simulink model "StampFly_IMU400"  (R2026b)
settings: Solver=FixedStepDiscrete  StopTime=inf  FixedStep=Official.Step
PostLoadFcn:
  | run(fullfile(fileparts(get_param('StampFly_IMU400','FileName')),'config','startup.m'));
InitFcn:
  | init_imu_flight;
undefined symbols (not defined in the file): Bottom, Official
libraries: slpidlib x7, simulink x4, mspfiltlib x1
(part 4 of 4)

== matlab function StampFly_IMU400/AttitudeAltitudeEstimation400/IMUAttitude400/FilterInputs ==
  data: rates input; accelMps2 output; accelG input; mode input; reset input; gyroRps output; run output; filterReset output
function [accelMps2,gyroRps,run,filterReset]=IMUFilterInputs(rates,accelG,mode,reset)
%IMUFILTERINPUTS Match the previous estimator axes and use gravity-positive NED.
%#codegen
% The previous Madgwick frame is [bodyY bodyX -bodyZ]. Its accelerometer
% vector has +g on Z at rest. NED IMU Filter uses the same gravity sign.
accelMps2=single([accelG(2),accelG(1),-accelG(3)])*single(9.80665);
gyroRps=single([rates(2),rates(1),-rates(3)]);
run=mode>uint8(1);
% A disabled subsystem does not execute its Reset port. Retain reset requests
% during calibration/hold and apply them before the next fusion update.
persistent pendingReset
if isempty(pendingReset),pendingReset=false;end
if reset,pendingReset=true;end
filterReset=pendingReset;
if run,pendingReset=false;end
end

== matlab function StampFly_IMU400/AttitudeAltitudeEstimation400/IMUAttitude400/FlightOutputs ==
  data: orientation input; angles output; angularVelocity input; run input; reset input; rawRates input; q output; rates output
function [angles,q,rates]=IMUFlightOutputs(orientation,angularVelocity,run,reset,rawRates)
%IMUFLIGHTOUTPUTS Preserve the previous estimator's flight-facing conventions.
%#codegen
% Match the previous angle/quaternion hold behavior before estimation starts.
% A reset clears orientation but retains the last angles until the next update.
persistent heldAngles heldQuaternion heldBias
if isempty(heldAngles)
    heldAngles=zeros(3,1,'single');
    heldQuaternion=single([1;0;0;0]);
    heldBias=zeros(3,1,'single');
end
if reset
    heldQuaternion=single([1;0;0;0]);
    heldBias=zeros(3,1,'single');
end
correctedRates=single([angularVelocity(2);angularVelocity(1);-angularVelocity(3)]);
if run
    heldQuaternion=single(orientation(:));
    w=heldQuaternion(1);x=heldQuaternion(2);y=heldQuaternion(3);z=heldQuaternion(4);
    roll=atan2(single(2)*(w*x+y*z),single(1)-single(2)*(x*x+y*y));
    pitch=asin(min(single(1),max(single(-1),single(2)*(w*y-z*x))));
    yaw=atan2(single(2)*(x*y+w*z),single(1)-single(2)*(y*y+z*z));
    % Retain the original rounded radians/degrees factors and yaw offset.
    heldAngles=[pitch*single(57.29578);roll*single(57.29578); ...
        -(yaw*single(57.29578)+single(180))]*single(pi/180);
    heldBias=single(rawRates(:))-correctedRates;
end
angles=heldAngles;q=heldQuaternion;
% Keep the live gyro path when fusion is disabled; the retained residual bias
% is zero during startup and after reset. No extra sample delay is introduced.
rates=single(rawRates(:))-heldBias;
if run,rates=correctedRates;end
end

== stateflow chart StampFly_IMU400/FlightControl400/TakeoffHoverControl400/FlightCommand400/TakeoffLandingCommand ==
  settings: description=|
      | 離陸・ホバリング・着陸の指令生成（400 Hz）
      | Parking: 高度0.5 m/推力0へ初期化。自動離陸: 0〜499周期は3.8 V基準、500〜999周期は実電圧トリム。
      | AutoHover: 1000周期後の基準推力。目標高度0.05〜1.8 m、スティックで更新。
      | ManualAltitude/AutoHover/Landingの遷移条件は図に表示。演算順・状態保持・AltFlag保持は公式互換。
      | Chart内にMATLAB関数は置かない。
  state CommandPhases [parallel]
    settings: executionOrder=1
    state Parking
      en: Base=single(0);Alt=single(.5);Counter=uint16(0);landingActive=false;AltFlag=false;
    state TakeoffReference
      en: ControlMode=uint8(stick(5));AltFlag=true;
      Base=min(single(Counter)/single(1000),(-single(.2448)*single(3.8)+single(1.5892)));Counter=Counter+uint16(1);
      th=stick(4);if th>-.2 && th<.2,th=single(0);end
      Alt=min(max(single(double(Alt)+double(th)*.001),single(.05)),single(1.8));
      if rangeFlag>RangeOld || rangeFlag==20,Base=Base-single(.02);RangeOld=rangeFlag;end
      raw=single(double(Base)*3.7);
    state ManualAltitude
      en: ControlMode=uint8(stick(5));manual=true;th=min(max(stick(4),single(0)),single(1));
      if th>-.2 && th<.2,th=single(0);end
      raw=single((.00413+double(single(3.3)*th-single(5.44)*th*th+single(3.13)*th*th*th))*3.7);
    state TakeoffBattery
      en: ControlMode=uint8(stick(5));AltFlag=true;
      Base=min(single(Counter)/single(1000),(-single(.2448)*voltage+single(1.5892)));Counter=Counter+uint16(1);
      th=stick(4);if th>-.2 && th<.2,th=single(0);end
      Alt=min(max(single(double(Alt)+double(th)*.001),single(.05)),single(1.8));
      if rangeFlag>RangeOld || rangeFlag==20,Base=Base-single(.02);RangeOld=rangeFlag;end
      raw=single(double(Base)*3.7);
    state AutoHover
      en: ControlMode=uint8(stick(5));AltFlag=true;
      Base=(-single(.2448)*voltage+single(1.5892));
      th=stick(4);if th>-.2 && th<.2,th=single(0);end
      Alt=min(max(single(double(Alt)+double(th)*.001),single(.05)),single(1.8));
      if rangeFlag>RangeOld || rangeFlag==20,Base=Base-single(.02);RangeOld=rangeFlag;end
      raw=single(double(Base)*3.7);
    state Landing
      en: AltFlag=false;
      if ~landingActive,landingActive=true;History(:)=height;Base=(-single(.2448)*voltage+single(1.5892));end
      if History(10)>=height,Base=single(double(Base)*.9999);end
      if height<.15,Base=single(double(Base)*.999);end
      if height<.1,landingActive=false;end
      for j=2:10,History(j)=History(j-1);end
      History(1)=height;
    state Hold
    CommandPhases -> (junction 50) : step
    (junction 50) -> AutoHover [order 6] : [mode==2 && uint8(stick(6))==4]
    (junction 50) -> Hold [order 7]
    (junction 50) -> Parking [order 1] : [mode==3]
    (junction 50) -> Landing [order 2] : [mode==5]
    (junction 50) -> TakeoffBattery [order 5] : [mode==2 && uint8(stick(6))==4 && Counter<1000]
    (junction 50) -> TakeoffReference [order 4] : [mode==2 && uint8(stick(6))==4 && Counter<500]
    (default) -> Hold : /{Alt=single(.5);Base=single(0);Counter=uint16(0);RangeOld=uint8(0);landingActive=false;History=zeros(10,1,'single');AltFlag=false;ControlMode=uint8(0);th=single(0);j=double(0);}
    (junction 50) -> ManualAltitude [order 3] : [mode==2 && uint8(stick(6))~=4]
  state CycleOutputs [parallel]
    en: raw=single(0);manual=false;
    send(step,CommandPhases);
    alt=Alt;base=Base;counter=Counter;auto=AltFlag;controlMode=single(ControlMode);
    du: raw=single(0);manual=false;
    send(step,CommandPhases);
    alt=Alt;base=Base;counter=Counter;auto=AltFlag;controlMode=single(ControlMode);
    settings: executionOrder=2
  note: 離陸・ホバリング・着陸の指令生成（400 Hz）
      | Parking: 高度0.5 m/推力0へ初期化。自動離陸: 0〜499周期は3.8 V基準、500〜999周期は実電圧トリム。
      | AutoHover: 1000周期後の基準推力。目標高度0.05〜1.8 m、スティックで更新。
      | ManualAltitude/AutoHover/Landingの遷移条件は図に表示。演算順・状態保持・AltFlag保持は公式互換。
      | Chart内にMATLAB関数は置かない。
  data: stick input single; height input single; voltage input single; rangeFlag input uint8; mode input uint8; alt output single; base output single; counter output uint16; raw output single; auto output boolean; manual output boolean; controlMode output single; Alt local single; Base local single; Counter local uint16; RangeOld local uint8; landingActive local boolean; History local single; AltFlag local boolean; ControlMode local uint8; th local single; j local double
  events: step local FUNCTION_CALL_EVENT

== matlab function StampFly_IMU400/LEDAndBuzzer400/StatusOutputs400/StatusIndicators400 ==
  data: arg_mode input uint8; arg_color1 output uint32; arg_controlMode input single; arg_altFlag input uint8; arg_lowVoltage input uint8; arg_rcError input uint8; arg_ahrsFlag input uint8; arg_button input uint8; arg_color2 output uint32; arg_tone output uint32; arg_restart output boolean
function [arg_color1,arg_color2,arg_tone,arg_restart]=stepFn(arg_mode,arg_controlMode,arg_altFlag,arg_lowVoltage,arg_rcError,arg_ahrsFlag,arg_button)
% 公式led_driveの状態色。ブザーの200ms待機は400Hzカウンターへ置換。
%#codegen
persistent Blink Rainbow C1 C2 Tick AHRSPrev ToneTicks ButtonCount WasPressed;
if isempty(Blink)
 Blink=uint16(0);Rainbow=uint32(255);C1=uint32(0);C2=uint32(0);Tick=uint16(0);AHRSPrev=uint8(0);ToneTicks=uint16(0);ButtonCount=uint8(0);WasPressed=false;
end
if arg_mode==1,C1=uint32(hex2dec('FF00FF'));C2=C1;
elseif arg_mode==5,C1=uint32(hex2dec('00FF00'));C2=C1;
elseif arg_mode==2
 c=uint32(hex2dec('FFFF00'));
 if arg_controlMode~=0,c=uint32(hex2dec('DC669B'));end
 if arg_altFlag>=1,c=uint32(hex2dec('331155'));end
 if arg_rcError==1,c=uint32(hex2dec('FF0000'));end
 C1=c;C2=c;if arg_lowVoltage>=100,C1=uint32(hex2dec('18EBF9'));end
elseif arg_mode==3
 if arg_lowVoltage<100
  if Blink==0
   top=bitand(Rainbow,uint32(hex2dec('800000')))~=0;Rainbow=bitshift(Rainbow,1);if top,Rainbow=bitor(Rainbow,uint32(1));end
   C1=Rainbow;C2=Rainbow;Blink=Blink+uint16(1);
  end
  Blink=Blink+uint16(1);if Blink>20,Blink=uint16(0);end
 else
  if Blink<10,C1=uint32(hex2dec('18EBF9'));C2=C1;
  elseif Blink<200,C1=uint32(0);C2=uint32(0);else,Blink=uint16(0);end
  Blink=Blink+uint16(1);
 end
 if arg_ahrsFlag~=AHRSPrev && arg_ahrsFlag==1,ToneTicks=uint16(80);end
 AHRSPrev=arg_ahrsFlag;
end
arg_tone=uint32(0);
% Startup notes from official buzzer.h. Four 200ms notes, then silence.
if Tick<320
 notes=uint32([294 441 350 393]);idx=min(floor(double(Tick)/80)+1,4);arg_tone=notes(idx);Tick=Tick+uint16(1);
elseif ToneTicks>0,arg_tone=uint32(4000);ToneTicks=ToneTicks-uint16(1);end
arg_restart=false;
if arg_button==1,ButtonCount=min(ButtonCount+uint8(1),uint8(40));if ButtonCount>=4,WasPressed=true;end
elseif WasPressed,arg_restart=true;WasPressed=false;ButtonCount=uint8(0);else,ButtonCount=uint8(0);end
% FastLED brightness15, show32: cap displayed channels without changing logic.
arg_color1=scale(C1);arg_color2=scale(C2);
end
function c=scale(x)
r=bitand(bitshift(x,-16),uint32(255));g=bitand(bitshift(x,-8),uint32(255));b=bitand(x,uint32(255));
c=bitor(bitor(bitshift(uint32(double(r)*15/255),16),bitshift(uint32(double(g)*15/255),8)),uint32(double(b)*15/255));
end

== matlab function StampFly_IMU400/FlightControl400/TakeoffHoverControl400/AltitudeControl400/SelectVerticalReference ==
  data: arg_zRef input single; arg_vRef output single; arg_mode input uint8; arg_auto input boolean
function arg_vRef=stepFn(arg_zRef,arg_mode,arg_auto)
% Auto高度補正が優先。公式else-ifの順序を維持。
%#codegen
arg_vRef=arg_zRef;if ~arg_auto && arg_mode==5,arg_vRef=single(-.15);end
end

== matlab function StampFly_IMU400/JoystickFeedback40/JoyStickTelemetry40/OfficialTelemetryValues ==
  data: arg_t input single; arg_values output single; arg_dt input single; arg_a input single; arg_r input single; arg_cd input single; arg_accel input single; arg_voltage input single; arg_duty input single; arg_z input single; arg_sd input single; arg_v input single
function arg_values=stepFn(arg_t,arg_dt,arg_a,arg_r,arg_cd,arg_accel,arg_voltage,arg_duty,arg_z,arg_sd,arg_v)
% 公式120byteテレメトリの27個のfloat。バイト送信は専用IOブロック。
%#codegen
arg_values=zeros(27,1,'single');arg_values(1:2)=[arg_t;arg_dt];arg_values(3:8)=[arg_a;arg_r]*single(180/pi);
arg_values(9:13)=arg_cd(6:10)*single(180/pi);arg_values(14)=single(double(arg_cd(5))/3.7);
arg_values(15)=arg_voltage;arg_values(16:18)=arg_accel([2 1 3])/single(9.80665);arg_values(18)=-arg_values(18);
arg_values(19:20)=[arg_v;arg_cd(4)];arg_values(21:22)=arg_duty(2:3);
arg_values(23:27)=[arg_cd(1);arg_z;arg_sd(3);arg_sd(1:2)];
end

== matlab function StampFly_IMU400/FlightControl400/TakeoffHoverControl400/AltitudeControl400/ThrustCorrectionLimits ==
  data: arg_arg_command input single; arg_arg_thrust output single; arg_arg_correction input single; arg_arg_base input single; arg_arg_auto input boolean; arg_arg_manual input boolean; arg_arg_velEnable input boolean; arg_branch input uint8; arg_arg_dt input single; arg_arg_oldFilter input single; arg_arg_lastThrust input single; arg_arg_filter output single; arg_arg_last output single
function [arg_arg_thrust,arg_arg_filter,arg_arg_last]=stepFn(arg_arg_command,arg_arg_correction,arg_arg_base,arg_arg_auto,arg_arg_manual,arg_arg_velEnable,arg_branch,arg_arg_dt,arg_arg_oldFilter,arg_arg_lastThrust)
% Auto correction takes priority over landing correction.
%#codegen
arg_arg_thrust=arg_arg_command;arg_arg_filter=arg_arg_oldFilter;
if arg_branch==3,arg_arg_filter=single(0);elseif arg_arg_manual,arg_arg_filter=arg_arg_command;end
if arg_arg_velEnable
 arg_arg_filter=filterStep(single(double(arg_arg_base+arg_arg_correction)*3.7),arg_arg_dt,single(.01),arg_arg_filter);arg_arg_thrust=arg_arg_filter;
 if arg_arg_auto
  if double(arg_arg_thrust)/3.7>double(single(arg_arg_base*single(1.15))),arg_arg_thrust=single(3.7*double(arg_arg_base)*double(single(1.15)));end
  if double(arg_arg_thrust)/3.7<double(single(arg_arg_base*single(.85))),arg_arg_thrust=single(3.7*double(arg_arg_base)*double(single(.85)));end
 end
end
if arg_branch==3,arg_arg_thrust=arg_arg_lastThrust;arg_arg_last=arg_arg_lastThrust;else,arg_arg_last=arg_arg_thrust;end
end
function s=filterStep(u,h,T,s),s=s*T/(T+h)+u*h/(T+h);end

== matlab function StampFly_IMU400/FlightControl400/TakeoffHoverControl400/AttitudeControl400/StickToAngleRate ==
  data: arg_arg_stick input single; arg_arg_angle output single; arg_branch input uint8; arg_arg_run input boolean; arg_arg_reset input boolean; arg_arg_lastRate input single; arg_arg_controlMode input single; arg_arg_directRate output single; arg_arg_resetError output single
function [arg_arg_angle,arg_arg_directRate,arg_arg_resetError]=stepFn(arg_arg_stick,arg_branch,arg_arg_run,arg_arg_reset,arg_arg_lastRate,arg_arg_controlMode)
% command、角度目標、中立点を別々に保持。Sportは角度commandを更新しない。
%#codegen
persistent Angle Centers AngleCmd YawCmd;
if isempty(Angle),Angle=zeros(2,1,'single');Centers=zeros(3,1,'single');AngleCmd=zeros(2,1,'single');YawCmd=single(0);end
arg_arg_directRate=arg_arg_lastRate;arg_arg_resetError=Angle;
commandCalled=arg_branch==2 || arg_branch==5;
if commandCalled
 if uint8(arg_arg_controlMode)==0 || arg_branch==5,AngleCmd=min(max(single(.4*double(arg_arg_stick(1:2))),single(-1)),single(1));end
 YawCmd=min(max(arg_arg_stick(3),single(-1)),single(1));
 arg_arg_directRate(3)=single(2*pi*double(YawCmd-Centers(3)));
 if uint8(arg_arg_controlMode)==1,arg_arg_directRate(1)=rateCommand(arg_arg_stick(1));arg_arg_directRate(2)=rateCommand(arg_arg_stick(2));end
end
if arg_arg_reset,Centers(1:2)=AngleCmd;end
if arg_arg_reset,Centers(3)=YawCmd;end
if arg_arg_run && uint8(arg_arg_controlMode)==0
 limit=single(30*pi/180);Angle=min(max(single(.5*pi*double(AngleCmd-Centers(1:2))),-limit),limit);
end
if arg_branch==3,arg_arg_directRate(1)=single(0);end
if arg_arg_reset,arg_arg_directRate(:)=single(0);end
arg_arg_angle=Angle;
end
function y=rateCommand(x)
x=min(max(x,single(-1)),single(1));a=abs(x);t=a*(a*a*a*a*a*single(.5)+a*single(.5));
y=single(pi/180)*((single(1600)-single(70))*t+single(70)*a);if x<0,y=-y;end
end

== matlab function StampFly_IMU400/FlightControl400/TakeoffHoverControl400/AttitudeControl400/SelectRateReference ==
  data: direct input single; rate output single; rollPID input single; pitchPID input single; angleEnable input boolean
function rate =stepFn(direct,rollPID,pitchPID,angleEnable)
% 日本語の説明はブロック注釈とDescriptionを参照。
%#codegen
            rate=direct;if angleEnable,rate(1)=rollPID;rate(2)=pitchPID;end
end

== matlab function StampFly_IMU400/FlightControl400/TakeoffHoverControl400/FlightDiagnostics400/ControlDiagnosticPack ==
  data: alt input single; diag output single; base input single; counter input uint16; zRef input single; thrust input single; angle input single; rate input single; rollTorque input single; pitchTorque input single; yawTorque input single; before input single
function diag =stepFn(alt,base,counter,zRef,thrust,angle,rate,rollTorque,pitchTorque,yawTorque,before)
% 日本語の説明はブロック注釈とDescriptionを参照。
%#codegen
            diag=[alt;base;single(counter);zRef;thrust;angle;rate;rollTorque;pitchTorque;yawTorque;before];
end

== stateflow chart StampFly_IMU400/FlightControl400/TakeoffHoverControl400/FlightCommand400/FinalizeFlightMode ==
  settings: description=Normal flight: finalize the mode; excessive acceleration and completed landing return to parking.
  state FinalModes [parallel]
    settings: executionOrder=1
    state OTHER
      en: mode=preMode;
    state INIT
      en: mode=uint8(0);
    state LANDING
      en: mode=uint8(5);
    state PARKING
      en: mode=uint8(3);
    state FLIGHT
      en: mode=uint8(2);
    state AVERAGE
      en: mode=uint8(1);
    (default) -> INIT
    (junction 27) -> OTHER [order 8]
    (junction 27) -> INIT [order 3] : [preMode==uint8(0)]
    FinalModes -> (junction 27) : decide
    (junction 27) -> AVERAGE [order 4] : [preMode==uint8(1)]
    (junction 27) -> LANDING [order 7] : [preMode==uint8(5)]
    (junction 27) -> FLIGHT [order 6] : [preMode==uint8(2)]
    (junction 27) -> PARKING [order 5] : [preMode==uint8(3)]
    (junction 27) -> PARKING [order 2] : [branch==5 && height<.1]
    (junction 27) -> PARKING [order 1] : [(branch==2 || branch==5) && overG==1]
  state CycleInput [parallel]
    en: mode=preMode;send(decide,FinalModes);
    du: mode=preMode;send(decide,FinalModes);
    settings: executionOrder=2
  note: Basic flight: takeoff, hover, landing and normal fault handling.
  data: branch input uint8; preMode input uint8; height input single; overG input uint8; mode output uint8
  events: decide local FUNCTION_CALL_EVENT

== matlab function StampFly_IMU400/FlightControl400/TakeoffHoverControl400/FlightCommand400/ControlGating400/ControlEnableReset ==
  data: arg_arg_raw input single; arg_arg_command output single; arg_arg_manual input boolean; arg_arg_auto input boolean; arg_branch input uint8; arg_arg_controlMode input single; arg_arg_dt input single; arg_arg_oldFilter input single; arg_arg_lastThrust input single; arg_arg_mode input uint8; arg_arg_run output boolean; arg_arg_reset output boolean; arg_arg_altEnable output boolean; arg_arg_angleEnable output boolean; arg_arg_velEnable output boolean
function [arg_arg_command,arg_arg_run,arg_arg_reset,arg_arg_altEnable,arg_arg_angleEnable,arg_arg_velEnable]=stepFn(arg_arg_raw,arg_arg_manual,arg_arg_auto,arg_branch,arg_arg_controlMode,arg_arg_dt,arg_arg_oldFilter,arg_arg_lastThrust,arg_arg_mode)
% Normal-flight enable/reset decisions and thrust filtering.
%#codegen
arg_arg_command=arg_arg_raw;
if arg_arg_manual,arg_arg_command=filterStep(arg_arg_raw,arg_arg_dt,single(.01),arg_arg_oldFilter);end
if arg_branch==5 || arg_branch==3,arg_arg_command=arg_arg_lastThrust;end
active=arg_branch==2 || arg_branch==5;
arg_arg_reset=active && double(arg_arg_command)/3.7<double(single(.1));
arg_arg_run=active && ~arg_arg_reset;
arg_arg_altEnable=arg_arg_run && arg_arg_auto;
arg_arg_angleEnable=arg_arg_run && uint8(arg_arg_controlMode)==0;
arg_arg_velEnable=arg_arg_run && (arg_arg_auto || arg_arg_mode==5);
end
function s=filterStep(u,h,T,s),s=s*T/(T+h)+u*h/(T+h);end

== matlab function StampFly_IMU400/SensorCorrection400/IMUBiasCalibration ==
  data: a input single; offset output single; g input single; mode input uint8; count output uint16
function [offset,count]=stepFn(a,g,mode)
% 日本語の説明はブロック注釈とDescriptionを参照。
%#codegen
persistent Offset Count;
if isempty(Offset)
Offset=zeros(4,1,'single');
Count=uint16(0);
end
            if mode==0,Offset(:)=single(0);Count=uint16(0);
            elseif mode==1 && Count<uint16(800)
                n=single(Count);
                Offset=(n*Offset+[g;a(3)])/(n+single(1));
                Count=Count+uint16(1);
            end
            offset=Offset;count=Count;
end

== matlab function StampFly_IMU400/SensorCorrection400/ToFHoldOutlierFilter ==
  data: mm input int16; alt output single; fresh input uint8; mode input uint8; dt input single; raw output int16
function [alt,raw]=stepFn(mm,fresh,mode,dt)
% 日本語の説明はブロック注釈とDescriptionを参照。
%#codegen
persistent History Range Raw Outlier Alt PreviousMode;
if isempty(History)
History=zeros(4,1,'int16');
Range=int16(0);
Raw=int16(0);
Outlier=uint8(0);
Alt=single(0);
PreviousMode=uint8(0);
end
            if mode==3 && mode~=PreviousMode,History(:)=int16(0);Alt=single(0);end
            if mode>1
                if fresh~=0
                    Raw=mm;if mm>int16(20),Range=mm;end
                    delta=int32(Range)-int32(History(2));
                    if abs(delta)>int32(500) && Outlier<uint8(2)
                        extrap=int32(History(2))+idivide(int32(History(2))-int32(History(4)),int32(2),'fix');
                        Range=int16(extrap);Outlier=Outlier+uint8(1);
                    else
                        Outlier=uint8(0);History(4)=History(3);History(3)=History(2);History(2)=Range;
                    end
                end
                Alt=filterStep(single(double(Range)/1000),dt,single(0.005),Alt);
            end
            alt=Alt;raw=Raw;PreviousMode=mode;
end

function s = filterStep(u,h,T,s)
%FILTERSTEP Exact Filter::update, including operation ordering.
%#codegen
s = s*T/(T+h) + u*h/(T+h);
end

== matlab function StampFly_IMU400/AttitudeAltitudeEstimation400/AltitudeKalman ==
  data: alt input single; height output single; az input single; mode input uint8; dt input single; parkingReset input boolean; velocity output single; bias output single
function [height,velocity,bias]=stepFn(alt,az,mode,dt,parkingReset)
% 日本語の説明はブロック注釈とDescriptionを参照。
%#codegen
persistent State First PreviousMode;
if isempty(State)
State=kalmanInitial();
First=false;
PreviousMode=uint8(0);
end
            if parkingReset,[~,State]=kalmanStep(single(0),single(0),dt,true,State);end
            if mode==3 && mode~=PreviousMode,First=false;end
            if mode>1
                if First,[~,State]=kalmanStep(alt,az,dt,false,State);else,First=true;end
            end
            velocity=State.output(1);height=State.output(2);bias=State.output(3);PreviousMode=mode;
end

function [y,s] = kalmanStep(z,acc,h,resetState,s)
%KALMANSTEP Direct translation of Alt_kalman::update, state [v;z;bias].
% Preserve reset(): covariance and public output reset, private x is retained.
%#codegen
if resetState
    s.P = single(100)*eye(3,'single'); s.output(:) = single(0);
else
    p=s.P; b=single(-0.01); f=single(1)+h*b;
    xp=[s.x(1)+(acc-s.x(3))*h;s.x(2)+s.x(1)*h;s.x(3)*f];
    pp=zeros(3,3,'single');
    pp(1,1)=p(1,1)-h*(p(3,1)+p(1,3))+h*h*p(3,3)+h*h*single(0.01);
    pp(1,2)=h*(p(1,1)-p(3,2))-h*h*p(3,1)+p(1,2);
    pp(1,3)=f*(p(1,3)-h*p(3,3));
    pp(2,1)=h*(p(1,1)-p(2,3))-h*h*p(1,3)+p(2,1);
    pp(2,2)=h*h*p(1,1)+h*(p(2,1)+p(1,2))+p(2,2);
    pp(2,3)=f*(p(2,3)+h*p(1,3));
    pp(3,1)=f*(p(3,1)-h*p(3,3));
    pp(3,2)=f*(p(3,2)+h*p(3,1));
    pp(3,3)=f*f*p(3,3)+h*h;
    k=[pp(1,2);pp(2,2);pp(3,2)]/(pp(2,2)+single(0.004*0.004));
    e=z-xp(2); s.x=xp+k*e; s.output=s.x;
    s.P(1,:)=pp(1,:)-k(1)*pp(2,:);
    s.P(2,:)=pp(2,:)*(single(1)-k(2));
    s.P(3,:)=-k(3)*pp(2,:)+pp(3,:);
end
y=s.output;
end

function s = kalmanInitial()
%#codegen
s = struct('x',zeros(3,1,'single'),'P',single(100)*eye(3,'single'), ...
    'output',zeros(3,1,'single'));
end

== matlab function StampFly_IMU400/AttitudeAltitudeEstimation400/SensorFlags ==
  data: arg_accel input single; arg_flags output uint8; arg_azd input single; arg_voltage input single; arg_mode input uint8; arg_altFlag input uint8; arg_height input single; arg_rawRange input int16; arg_dt input single; arg_parkingReset input boolean
function arg_flags =stepFn(arg_accel,arg_azd,arg_voltage,arg_mode,arg_altFlag,arg_height,arg_rawRange,arg_dt,arg_parkingReset)
% 日本語の説明はブロック注釈とDescriptionを参照。
%#codegen
persistent Norm Voltage OverG RangeFlag LowVoltage PreviousMode;
if isempty(Norm)
Norm=single(0);
Voltage=single(0);
OverG=uint8(0);
RangeFlag=uint8(0);
LowVoltage=uint8(0);
PreviousMode=uint8(0);
end
            if arg_parkingReset,OverG=uint8(0);RangeFlag=uint8(0);end
            if arg_mode==3 && arg_mode~=PreviousMode,Norm=single(0);end
            if arg_mode>1
                if (arg_height>single(2) && arg_altFlag~=0) || arg_rawRange==0,RangeFlag=min(RangeFlag+uint8(1),uint8(20));else,RangeFlag=uint8(0);end
            end
            normA=sqrt(arg_accel(1)*arg_accel(1)+arg_accel(2)*arg_accel(2)+arg_azd*arg_azd);
            Norm=filterStep(normA,arg_dt,single(.005),Norm);
            if Norm>single(2),OverG=uint8(1);end
            Voltage=filterStep(arg_voltage,arg_dt,single(.005),Voltage);
            if LowVoltage~=uint8(100)
                if Voltage<single(3.34),LowVoltage=LowVoltage+uint8(1);else,LowVoltage=uint8(0);end
                LowVoltage=min(LowVoltage,uint8(100));
            end
            arg_flags=[OverG;RangeFlag;LowVoltage];PreviousMode=arg_mode;
end

function s = filterStep(u,h,T,s)
%FILTERSTEP Exact Filter::update, including operation ordering.
%#codegen
s = s*T/(T+h) + u*h/(T+h);
end

== stateflow chart StampFly_IMU400/OfficialFlightSupervisor ==
  settings: description=|
      | 飛行モードの状態遷移図（400 Hz）
      | INIT→AVERAGE→PARKING→FLIGHT→LANDING。通信途絶・OverG・ボタンを遷移条件で判断。
      | CycleInputsが1周期分の入力を整理し、syncで前周期の確定状態に同期、decideで今回の遷移を実行。
      | branchは今回の分岐開始状態、modeは今回の判断後の状態。MATLAB関数はChart内に置かない。
  state FlightModes [parallel]
    settings: executionOrder=1
    state PARKING
      en: mode=uint8(3);
    state AVERAGE
      en: mode=uint8(1);
    state INIT
      en: mode=uint8(0);
    state FLIGHT
      en: mode=uint8(2);
    state LANDING
      en: mode=uint8(5);
    state OTHER
      en: mode=branch;
    (default) -> INIT : /{calibration=uint16(0); buttonCounter=int8(0); buttonState=uint8(0); chatter=uint8(0); lastAHRS=uint8(0); connectionCounter=uint16(0); buttonEvent=false; calibrationDone=false;}
    AVERAGE -> PARKING : decide[calibrationDone]
    INIT -> AVERAGE : decide
    (junction 43) -> AVERAGE [order 2] : [branch==uint8(1)]
    (junction 43) -> INIT [order 1] : [branch==uint8(0)]
    PARKING -> FLIGHT : decide[buttonEvent]/{ahrsReset=true;}
    FLIGHT -> PARKING [order 1] : decide[flags(1)==1]/{ahrsReset=true;}
    (junction 43) -> PARKING [order 3] : [branch==uint8(3)]
    LANDING -> PARKING : decide[buttonEvent]
    FLIGHT -> LANDING [order 2] : decide[buttonEvent || connected==0]/{ahrsReset=true;}
    (junction 43) -> LANDING [order 5] : [branch==uint8(5)]
    (junction 43) -> FLIGHT [order 4] : [branch==uint8(2)]
    FlightModes -> (junction 43) : sync
    (junction 43) -> OTHER [order 6]
  state CycleInputs [parallel]
    en: branch=previousMode; mode=branch; ahrsReset=false; parkingReset=branch==3;
    buttonEvent=false; calibrationDone=false;
    if newPacket~=0, connectionCounter=uint16(0); end
    connected=uint8(connectionCounter<uint16(40));
    if branch==1
    calibrationDone=calibration>=uint16(800);
    if ~calibrationDone, calibration=calibration+uint16(1); end
    elseif branch~=0
    if button==1
    buttonCounter=buttonCounter+int8(1);
    if buttonCounter>int8(10),buttonCounter=int8(10);buttonState=uint8(1);end
    else
    buttonCounter=buttonCounter-int8(1);
    if buttonCounter<int8(-10),buttonCounter=int8(-10);buttonState=uint8(0);end
    end
    if chatter==0
    if buttonState==1,chatter=uint8(1);end
    elseif buttonState==0
    chatter=chatter+uint8(1);
    if chatter>uint8(40),chatter=uint8(0);buttonEvent=true;end
    end
    if branch==3
    if ahrsFlag~=lastAHRS
    if ahrsFlag==1,ahrsReset=true;end
    lastAHRS=ahrsFlag;
    end
    elseif branch==2
    connectionCounter=uint16(mod(double(connectionCounter)+1,65536));
    connected=uint8(connectionCounter<uint16(40));
    end
    end
    send(sync,FlightModes);
    send(decide,FlightModes);
    du: branch=previousMode; mode=branch; ahrsReset=false; parkingReset=branch==3;
    buttonEvent=false; calibrationDone=false;
    if newPacket~=0, connectionCounter=uint16(0); end
    connected=uint8(connectionCounter<uint16(40));
    if branch==1
    calibrationDone=calibration>=uint16(800);
    if ~calibrationDone, calibration=calibration+uint16(1); end
    elseif branch~=0
    if button==1
    buttonCounter=buttonCounter+int8(1);
    if buttonCounter>int8(10),buttonCounter=int8(10);buttonState=uint8(1);end
    else
    buttonCounter=buttonCounter-int8(1);
    if buttonCounter<int8(-10),buttonCounter=int8(-10);buttonState=uint8(0);end
    end
    if chatter==0
    if buttonState==1,chatter=uint8(1);end
    elseif buttonState==0
    chatter=chatter+uint8(1);
    if chatter>uint8(40),chatter=uint8(0);buttonEvent=true;end
    end
    if branch==3
    if ahrsFlag~=lastAHRS
    if ahrsFlag==1,ahrsReset=true;end
    lastAHRS=ahrsFlag;
    end
    elseif branch==2
    connectionCounter=uint16(mod(double(connectionCounter)+1,65536));
    connected=uint8(connectionCounter<uint16(40));
    end
    end
    send(sync,FlightModes);
    send(decide,FlightModes);
    settings: executionOrder=2
  note: 飛行モードの状態遷移図（400 Hz）
      | INIT→AVERAGE→PARKING→FLIGHT→LANDING。通信途絶・OverG・ボタンを遷移条件で判断。
      | CycleInputsが1周期分の入力を整理し、syncで前周期の確定状態に同期、decideで今回の遷移を実行。
      | branchは今回の分岐開始状態、modeは今回の判断後の状態。MATLAB関数はChart内に置かない。
  data: previousMode input uint8; button input uint8; newPacket input uint8; flags input uint8; ahrsFlag input uint8; branch output uint8; mode output uint8; ahrsReset output boolean; parkingReset output boolean; connected output uint8; calibration local uint16; buttonCounter local int8; buttonState local uint8; chatter local uint8; lastAHRS local uint8; connectionCounter local uint16; buttonEvent local boolean; calibrationDone local boolean
  events: sync local FUNCTION_CALL_EVENT; decide local FUNCTION_CALL_EVENT
